simulink library "WECSim_Lib_Body_Elements"  (R2020b)
settings: Solver=VariableStepAuto  StartTime=0.0  StopTime=10.0  RelTol=1e-3
undefined symbols (not defined in the file or in its folder): body, simu, waves, X, Y, Z
libraries: nesl_utility x22, sm_lib x16, $bdroot x9, vrlib x3
(part 3 of 5)

== system WECSim_Lib_Body_Elements/Rigid Body/Hydrodynamic Body/B2B Subsystem/B2B ==
  CrossCoupling : Subsystem  mask{body=body}
      mask prompts: body "Body Number"
      mask help: This is used to
      mask init:
      | %In the initialization tab we place the code modifying the block
      | 
      | cb = gcb;
      | % position of initial blocks
      | set_param([cb '/vel1'],'Position',[200 1*50 240 (1*50+30)])
      | set_param([cb '/Mux1'], 'Position',[375 40 380 90])
      | set_param([cb '/vel'], 'Position',[410 59 440 71])
      | set_param([cb '/acc1'],'Position',[600 1*50 640 (1*50+30)])
      | set_param([cb '/Mux2'], 'Position',[775 40 780 90])
      | set_param([cb '/acc'], 'Position',[810 59 840 71])
      | set_param([cb '/Transport Delay1'], 'Position', [650 1*50 690 (1*50+30)])
      | 
      | % add/delete lines & blocks
      | newInputs = 0;
      | numbodies = body.total;
      | iBod = 2;
      | while iBod < 100
      |     try 
      |         find_system([cb,'/vel',num2str(iBod)],'Type','Block');
      |         if iBod > numbodies
      |             %delete 'From' blocks and lines if bodynumber > total bodies
      |             delete_line(cb,['vel',num2str(iBod),'/1'],['Mux',num2str(1),'/',num2str(iBod)])
      |             delete_line(cb,['acc',num2str(iBod),'/1'],['Transport Delay',num2str(iBod),'/1'])
      |             delete_line(cb,['Transport Delay',num2str(iBod),'/1'],['Mux',num2str(2),'/',num2str(iBod)])
      |             delete_block([cb '/vel',num2str(iBod)])
      |             delete_block([cb '/acc',num2str(iBod)])
      |             delete_block([cb '/Transport Delay',num2str(iBod)])
      |         end
      |     catch
      |         %set number of outputs for 'Mux Creator' blocks 
      |         if newInputs==0
      |             set_param([cb,'/Mux1'],'Inputs',num2str(numbodies))
      |             set_param([cb,'/Mux2'],'Inputs',num2str(numbodies))
      |         end
      |         if iBod <= numbodies
      |             newInputs = newInputs + 1;
      |             %add velocity 'From' block
      |             add_block('simulink/Signal Routing/From', [cb,'/vel',num2str(iBod)],'MakeNameUnique', 'on',...
      |             'Position',[200 iBod*50 240 (iBod*50+30)], 'BackgroundColor','green')
      |             h=[cb,'/vel',num2str(iBod)];
      |             responseName=['vel' num2str(iBod)];
      |             set_param(h,'GotoTag',responseName);
      |             %add acceleration 'From' block
      |             add_block('simulink/Signal Routing/From', [cb,'/acc',num2str(iBod)],'MakeNameUnique', 'on',...
      |             'Position',[600 iBod*50 640 (iBod*50+30)], 'BackgroundColor','green')
      |             h=[cb,'/acc',num2str(iBod)];
      |             responseName=['acc' num2str(iBod)];
      |             set_param(h,'GotoTag',responseName);
      |             % add transport delay block 
      |             add_block('simulink/Continuous/Transport Delay', [cb,'/Transport Delay',num2str(iBod)],'MakeNameUnique', 'on',...
      |             'Position',[650 iBod*50 690 (iBod*50+30)])
      |             h=[cb,'/Transport Delay',num2str(iBod)];
      |             set_param(h,'DelayTime',num2str(10e-8));
      |             %add lines
      |             add_line(cb,['vel',num2str(iBod),'/1'],['Mux',num2str(1),'/',num2str(iBod)])
      |             add_line(cb,['acc',num2str(iBod),'/1'],['Transport Delay',num2str(iBod),'/1'])
      |             add_line(cb,['Transport Delay',num2str(iBod),'/1'],['Mux',num2str(2),'/',num2str(iBod)])
      |             
      |         else
      |             break
      |         end
      |     end
      |     iBod = iBod + 1;
      | end
      mask Callback body: %customsat_callback('input',gcb)
      mask DialogControl DescGroupVar Prompt: Coupling Block
      mask DialogControl DescTextVar Prompt: This block transfers the velocity and acceleration vectors between bodies allowing for the coupled hydrodynamic forces to be calculated.  This block should not be included if there is only one body or if the hydrodynamic coupling parameter is set to 'No' in the rigid body block.
  vel : Outport
  acc : Outport  Port=2
  wires:
  CrossCoupling/1(vel) -> vel/1
  CrossCoupling/2(acc) -> acc/1

== system WECSim_Lib_Body_Elements/Rigid Body/Hydrodynamic Body/B2B Subsystem/noB2B ==
  vel_in : Inport
  acc_in : Inport  Port=2
  vel : Outport
  acc : Outport  Port=2
  wires:
  vel_in/1 -> vel/1  "x"
  acc_in/1 -> acc/1

== system WECSim_Lib_Body_Elements/Rigid Body/Hydrodynamic Body/Hydrostatic Restoring Force Calculation/Linear and Nonlinear Restoring Force Variant Subsystem ==
  note: If simu.nlHydro == 0, use the linear force option.
      | If simu.nlHydro > 0, use the nonlinear force option.
  note: 1) Add Subsystem or Model blocks as valid variant choices.
      | 2) You cannot connect blocks at this level. At simulation, connectivity is automatically
      | determined, based on the active variant and port name matching.
  In1 : Inport
  In2 : Inport  Port=2
  Linear Hydrostatic Restoring Force : Subsystem  VariantControl=sv_b1_linearHydro
  Nonlinear Hydrostatic Restoring Force : Subsystem  VariantControl=sv_b1_nonlinearHydro
  Out1 : Outport

== system WECSim_Lib_Body_Elements/Rigid Body/Hydrodynamic Body/Morison Element and Viscous Damping Force Calculation/Morison Element Variant Subsystem ==
  note: If body.morisonElement.option == 0, Morison element is off and the Morison force is 0
      | If body.morisonElement.option == 1 | 2, Morison element is on
  note: 1) Add Subsystem or Model blocks as valid variant choices.
      | 2) You cannot connect blocks at this level. At simulation, connectivity is automatically
      | determined, based on the active variant and port name matching.
  displacement : Inport
  velocity : Inport  Port=2
  acceleration : Inport  Port=3
  time : Inport  Port=4
  Morison Element Off : Subsystem  VariantControl=sv_b1_MEOff
  Morison Element On : Subsystem  Variant=on  VariantControl=sv_b1_MEOn
  morison_force : Outport

== system WECSim_Lib_Body_Elements/Rigid Body/Hydrodynamic Body/Nonlinear Wave Elevation/Linear or Instantaneous Free Surface ==
  note: If simu.nlHydro < 2, use the mean water free surface.
      | If simu.nlHydro == 2, use the instantaneous water free surface
  note: 1) Add Subsystem or Model blocks as valid variant choices.
      | 2) You cannot connect blocks at this level. At simulation, connectivity is automatically
      | determined, based on the active variant and port name matching.
  In1 : Inport
  In2 : Inport  Port=2
  Instantaneous Water Free Surface : Subsystem  VariantControl=sv_b1_instFS
  Mean Water Free Surface : Subsystem  VariantControl=sv_b1_meanFS
  Out1 : Outport

== system WECSim_Lib_Body_Elements/Rigid Body/Hydrodynamic Body/Structure/Motion Sensor ==
  note: Measures the position, velocity, and acceleration of the follower (F) frame relative to the base (B) frame.
      | Ouputs a bus of 3 signals, each signal is a vector length 6.
  Bus Creator : BusCreator  Inputs=3
  Mux : Mux
  Mux1 : Mux  Inputs=6
  Mux2 : Mux  Inputs=6
  PS-Simulink Converter{,1..15} (16 alike) : nesl_utility/PS-Simulink Converter  PhysicalDomain=network_engine_domain  SubClassName=ps_output  LeftPortType=input  RightPortType=output  PseudoPeriodic=off  Frequencies=[]  VectorFormat=1-D array  Unit=1  AffineConversion=off
  Transform Sensor : sm_lib/Frames and Transforms/Transform Sensor  MeasurementFrame=World  RotationSequence=XYX  SenseAngle=off  SenseAxis=off  SenseQ=on  SenseR=off  SenseRotationSequence=off  SenseOmegaX=on  SenseOmegaY=on  SenseOmegaZ=on  SenseOmega=off  SenseQDot=off  SenseRDot=off  SenseRotationSequenceDot=off  SenseAlphaX=on  SenseAlphaY=on  SenseAlphaZ=on  SenseAlpha=off  SenseQDDot=off  SenseRDDot=off  SenseX=on  SenseY=on  SenseZ=on  SenseXYZ=off  SenseRad=off  SenseAzim=off  SenseDist=off  SenseInc=off  SenseXDot=on  SenseYDot=on  SenseZDot=on  SenseXYZDot=off  SenseRadDot=off  SenseAzimDot=off  SenseDistDot=off  SenseIncDot=off  SenseXDDot=on  SenseYDDot=on  SenseZDDot=on  SenseXYZDDot=off  SenseRadDDot=off  SenseAzimDDot=off  SenseDistDDot=off  SenseIncDDot=off
  quaternion2EulXYZ : MATLAB Function  TreatAsAtomicUnit=on
  F : PMIOPort  Side=Right
  B : PMIOPort  Port=2  Side=Left
  Response : Outport
  wires:
  Bus Creator/1 -> Response/1
  PS-Simulink Converter15/1 -> Mux2/3  "az"
  PS-Simulink Converter3/1 -> Mux1/6  "omegaz"
  PS-Simulink Converter11/1 -> Mux1/2  "vy"
  PS-Simulink Converter2/1 -> Mux1/5  "omegay"
  PS-Simulink Converter1/1 -> Mux1/4  "omegax"
  PS-Simulink Converter6/1 -> Mux2/6  "alphaz"
  PS-Simulink Converter5/1 -> Mux2/5  "alphay"
  PS-Simulink Converter9/1 -> Mux/3  "z"
  PS-Simulink Converter8/1 -> Mux/2  "y"
  PS-Simulink Converter7/1 -> Mux/1  "x"
  Mux2/1 -> Bus Creator/3  "acc"
  Mux1/1 -> Bus Creator/2  "vel"
  Mux/1 -> Bus Creator/1  "disp"
  PS-Simulink Converter14/1 -> Mux2/2  "ay"
  PS-Simulink Converter13/1 -> Mux2/1  "ax"
  PS-Simulink Converter12/1 -> Mux1/3  "vz"
  PS-Simulink Converter10/1 -> Mux1/1  "vx"
  PS-Simulink Converter4/1 -> Mux2/4  "alphax"
  quaternion2EulXYZ/1(E) -> Mux/4
  PS-Simulink Converter/1 -> quaternion2EulXYZ/1(Q)
  connections:
  B/RConn1 -- Transform Sensor/LConn1
  Transform Sensor/RConn1 -- F/RConn1
  PS-Simulink Converter15/LConn1 -- Transform Sensor/RConn17
  Transform Sensor/RConn2 -- PS-Simulink Converter/LConn1
  PS-Simulink Converter1/LConn1 -- Transform Sensor/RConn3
  Transform Sensor/RConn4 -- PS-Simulink Converter2/LConn1
  PS-Simulink Converter3/LConn1 -- Transform Sensor/RConn5
  Transform Sensor/RConn6 -- PS-Simulink Converter4/LConn1
  PS-Simulink Converter5/LConn1 -- Transform Sensor/RConn7
  Transform Sensor/RConn8 -- PS-Simulink Converter6/LConn1
  PS-Simulink Converter7/LConn1 -- Transform Sensor/RConn9
  Transform Sensor/RConn10 -- PS-Simulink Converter8/LConn1
  PS-Simulink Converter9/LConn1 -- Transform Sensor/RConn11
  PS-Simulink Converter10/LConn1 -- Transform Sensor/RConn12
  Transform Sensor/RConn13 -- PS-Simulink Converter11/LConn1
  PS-Simulink Converter12/LConn1 -- Transform Sensor/RConn14
  PS-Simulink Converter13/LConn1 -- Transform Sensor/RConn15
  Transform Sensor/RConn16 -- PS-Simulink Converter14/LConn1

== system WECSim_Lib_Body_Elements/Rigid Body/Hydrodynamic Body/Variable Hydrodynamics Control/Variable Hydrodynamics Subsystem ==
  note: 1) Add Subsystem or Model blocks as valid variant choices.
      | 2) You cannot connect blocks at this level. At simulation, connectivity is automatically
      | determined, based on the active variant and port name matching.
  all_hydroForce : Inport
  noVariableHydro : Subsystem  VariantControl=sv_b1_noVariableHydro
  variableHydro : Subsystem  VariantControl=sv_b1_variableHydro  mask{body=body}
      mask prompts: body "Body Number:"
      mask init: same as WECSim_Lib_Body_Elements/Flex Body/Variable Hydrodynamics Control/Variable Hydrodynamics Subsystem/variableHydro
  selected_hydroForce : Outport

== system WECSim_Lib_Body_Elements/Rigid Body/Hydrodynamic Body/Wave Diffraction and Excitation Force Calculation/FexcInputs ==
  Time : Inport
  Displacement : Inport  Port=2
  WaveElv : Inport  Port=3
  body_hydroForce : Inport  Port=4
  Out1 : Outport
  Out2 : Outport  Port=2
  Out3 : Outport  Port=3
  Out4 : Outport  Port=4
  wires:
  WaveElv/1 -> Out3/1
  Time/1 -> Out1/1
  Displacement/1 -> Out2/1
  body_hydroForce/1 -> Out4/1

== system WECSim_Lib_Body_Elements/Rigid Body/Hydrodynamic Body/Wave Diffraction and Excitation Force Calculation/Linear Wave Excitation Force Variant Subsystem ==
  note: No wave includes wave.type == 'noWave' or 'noWaveCIC'
      | Regular wave includes wave.type == 'regular' or 'regularCIC'
      | Irregular wave includes wave.type == 'irregular' or 'spectrumImport'
  note: 1) Add Subsystem or Model blocks as valid variant choices.
      | 2) You cannot connect blocks at this level. At simulation, connectivity is automatically
      | determined, based on the active variant and port name matching.
  Time : Inport
  Displacement : Inport  Port=2
  body_hydroForce : Inport  Port=3
  Irregular Wave Excitation Force : Subsystem  VariantControl=sv_irregularWaves_b1
  Irregular Wave NonLinearYaw : Subsystem  VariantControl=sv_irregularWavesYaw_b1
  Irregular Wave Full Direction : Subsystem  VariantControl=sv_fullDirIrregularWaves_b1
  No Wave Excitation Force : Subsystem  VariantControl=sv_noWave
  Regular Wave Excitation Force : Subsystem  VariantControl=sv_regularWaves_b1
  Regular Wave NonLinear Yaw : Subsystem  VariantControl=sv_regularWavesYaw_b1
  User Defined Wave Excitation Force : Subsystem  VariantControl=sv_udfWaves
  Linear Excitation : Outport

== system WECSim_Lib_Body_Elements/Rigid Body/Hydrodynamic Body/Wave Diffraction and Excitation Force Calculation/Nonlinear FK Force Variant Subsystem ==
  note: If simu.nlHydro == 0, use No Nonlinear FroudeKrylov force option (nonlinear force is zero),
      | If simu.nlHydro > 0, use the Nonlinear FroudeKrylov force option,
  note: 1) Add Subsystem or Model blocks as valid variant choices.
      | 2) You cannot connect blocks at this level. At simulation, connectivity is automatically
      | determined, based on the active variant and port name matching.
  Time : Inport
  Displacement : Inport  Port=2
  WaveElv : Inport  Port=3
  No Nonlinear FroudeKrylov Force : Subsystem  VariantControl=sv_b1_linearHydro
  With Nonlinear FroudeKrylov Force : Subsystem  TreatAsAtomicUnit=on  SystemSampleTime=simu.nonlinearDt  VariantControl=sv_b1_nonlinearHydro
  Nonlinear Excitation : Outport

== system WECSim_Lib_Body_Elements/Rigid Body/Hydrodynamic Body/Wave Diffraction and Excitation Force Calculation/Ramp function ==
  note: The ramp function R, is a smooth function:
      | R = (sin(3*pi/2 + pi * t/Tr) + 1)/2 from t=0 to t=Tr
  Time : Inport
  Add1 : Sum
  Add2 : Sum
  Constant1 : Constant  Value=1/2
  Constant2 : Constant
  Constant3 : Constant  Value=3*pi/2
  Constant4 : Constant  Value=pi
  Divide : Product  Inputs=*/
  Product1 : Product
  Product2 : Product
  Ramp Time : Constant  Value=simu.rampTime
  Sine Wave Function : Sin  TimeSource=Use external signal  SampleTime=0
  R : Outport
  wires:
  Constant1/1 -> Product1/2
  Sine Wave Function/1 -> Add1/2
  Time/1 -> Product2/1
  Product2/1 -> Add2/1
  Add2/1 -> Sine Wave Function/1
  Constant4/1 -> Divide/1
  Add1/1 -> Product1/1
  Divide/1 -> Product2/2  "frequency"
  Ramp Time/1 -> Divide/2  "t_ramp"
  Constant3/1 -> Add2/2  "phase"
  Constant2/1 -> Add1/1
  Product1/1 -> R/1

== system WECSim_Lib_Body_Elements/Rigid Body/Hydrodynamic Body/Wave Diffraction and Excitation Force Calculation/Second Order Excitation Force Variant Subsystem ==
  note: 1) Add Subsystem or Model blocks as valid variant choices.
      | 2) You cannot connect blocks at this level. At simulation, connectivity is automatically
      | determined, based on the active variant and port name matching.
  Time : Inport
  body_hydroForce : Inport  Port=2
  displacement : Inport  Port=3
  No Second Order Excitation Force : Subsystem  VariantControl=sv_b1_noSecondOrderExt
  With Second Order Excitation Force : Subsystem  VariantControl=sv_b1_secondOrderExt
  Second Order Excitation : Outport

== system WECSim_Lib_Body_Elements/Rigid Body/Hydrodynamic Body/Wave Radiation Forces Calculation/SS CI and Constant-Damping-CoeVariant Subsystem ==
  note: If the wave type is 'noWave' or 'regular' use constant coefficients.
      | If another wave type and simu.Calc ~= 1, use convolution integral calculation
      | If another wave type and simu.Calc == 1, use the state space calculation
      | If another wave type and simu.FIR == 1, use the FIR filter calculation
  note: 1) Add Subsystem or Model blocks as valid variant choices.
      | 2) You cannot connect blocks at this level. At simulation, connectivity is automatically
      | determined, based on the active variant and port name matching.
  velocity : Inport
  Constant Coefficients : Subsystem  VariantControl=sv_constantCoeff
  Convolution Integral Calculation : Subsystem  VariantControl=sv_convolution
  FIR Filter Calculation : Subsystem  VariantControl=sv_FIR
  "State-Space Calculation " : Subsystem  VariantControl=sv_stateSpace
  Out1 : Outport

== system WECSim_Lib_Body_Elements/Rigid Body/Hydrodynamic Body/Yaw Kinematic Transforms/No B2B ==
  note: If body.yaw.option == 1, interpolate the BEM coefficients to account for the effective change in the incoming wave direction.
  dispGlobal : Inport
  velGlobal : Inport  Port=2
  accGlobal : Inport  Port=3
  Constant : Constant  Value=body.yaw.option
  Yaw Kinematic Transforms : MATLAB Function  TreatAsAtomicUnit=on
  dispLoc : Outport
  velLoc : Outport  Port=2
  accLoc : Outport  Port=3
  wires:
  dispGlobal/1 -> Yaw Kinematic Transforms/2(dispGlobal)
  velGlobal/1 -> Yaw Kinematic Transforms/3(velGlobal)
  accGlobal/1 -> Yaw Kinematic Transforms/4(accGlobal)
  Constant/1 -> Yaw Kinematic Transforms/1(yaw)
  Yaw Kinematic Transforms/2(velLoc) -> velLoc/1
  Yaw Kinematic Transforms/1(dispLoc) -> dispLoc/1
  Yaw Kinematic Transforms/3(accLoc) -> accLoc/1

== system WECSim_Lib_Body_Elements/Rigid Body/Hydrodynamic Body/Yaw Kinematic Transforms/With B2B ==
  note: If body.yaw.option == 1, interpolate the BEM coefficients to account for the effective change in the incoming wave direction.
  dispGlobal : Inport
  velGlobal : Inport  Port=2
  accGlobal : Inport  Port=3
  Constant : Constant  Value=body.yaw.option
  Yaw Kinematic Transforms : MATLAB Function  TreatAsAtomicUnit=on
  dispLoc : Outport
  velLoc : Outport  Port=2
  accLoc : Outport  Port=3
  wires:
  Constant/1 -> Yaw Kinematic Transforms/1(yaw)
  Yaw Kinematic Transforms/1(dispLoc) -> dispLoc/1
  Yaw Kinematic Transforms/2(velLoc) -> velLoc/1
  Yaw Kinematic Transforms/3(accLoc) -> accLoc/1
  dispGlobal/1 -> Yaw Kinematic Transforms/2(dispGlobal)
  velGlobal/1 -> Yaw Kinematic Transforms/3(velGlobal)
  accGlobal/1 -> Yaw Kinematic Transforms/4(accGlobal)

== system WECSim_Lib_Body_Elements/Flex Body/Hydrostatic Restoring Force Calculation/Hydrostatic Restoring Force Calculation/Linear and Nonlinear Restoring Force Variant Subsystem/Linear Hydrostatic Restoring Force ==
  note: The total hydrostatic restoring force is due to a linear stiffness, the vertical buoyancy force (gravity - buoyancy) and a rotational buoyancy force if the center of gravity is not aligned with the center of buoyancy.
      |
      | F_restoring = F_linearRestoringStiffness + F_NetBuoyancy
      |
      | F_linear restoring = hydrostatic restoring coefficient * displacement
      | F_NetBuoyancy = F_gravity - F_buoyancy + F_rotational_buoyancy
      |
      | F_rotational_buoyancy = (cb-cg) x F_buoyancy
      | F_buoyancy = rho*g*V_0
      | F_gravity = m*g
  In1 : Inport
  Add : Sum
  Bus Selector1 : BusSelector  OutputSignals=mass,volume,centerBuoyancy,linearHydroRestCoef
  Net Buoyancy Force : Subsystem
  Product2 : Product  Multiplication=Matrix(*)
  Out1 : Outport
  wires:
  Net Buoyancy Force/1(F_NetBuoyancy) -> Add/1  "Net buoyancy force"
  Bus Selector1/1 -> Net Buoyancy Force/1(Body Mass)  "<mass>"
  Bus Selector1/4 -> Product2/1  "<linearHydroRestCoef>"
  Bus Selector1/2 -> Net Buoyancy Force/2(Volume)  "<volume>"
  [body1_hydroForce] -> Bus Selector1/1
  Bus Selector1/3 -> Net Buoyancy Force/3(Center of Buoyancy)  "<centerBuoyancy>"
  Product2/1 -> Add/2  "Linear Restoring Force"
  In1/1 -> Product2/2  "x"
  Add/1 -> Out1/1  "F_Restoring"

== system WECSim_Lib_Body_Elements/Flex Body/Hydrostatic Restoring Force Calculation/Hydrostatic Restoring Force Calculation/Linear and Nonlinear Restoring Force Variant Subsystem/Nonlinear Hydrostatic Restoring Force ==
  In1 : Inport
  In2 : Inport  Port=2
  Add : Sum
  Bus Selector1 : BusSelector  OutputSignals=storage.mass,volume,centerBuoyancy,linearHydroRestCoef
  Center of Gravity : Constant  Value=body.centerGravity
  Gravity : Constant  Value=simu.gravity
  Mux1 : Mux  Inputs=2
  Net Buoyancy Force : Subsystem
  Product2 : Product  Multiplication=Matrix(*)
  Rate Transition : RateTransition
  Rate Transition1 : RateTransition
  Restoring Forces : MATLAB Function  TreatAsAtomicUnit=on  SystemSampleTime=simu.nonlinearDt
  STL areas : Constant  Value=body.geometry.area
  STL centers : Constant  Value=body.geometry.center
  STL normal vectors : Constant  Value=body.geometry.norm
  Selector : Selector  InputPortWidth=body.dof  IndexOptions=Index vector (dialog)  Indices=[7:body.dofEnd]  OutputSizes=1
  To Workspace1 : ToWorkspace  VariableName=body1_hspressure_out  SaveFormat=Structure With Time  SampleTime=-1
      settings: Decimation=round(simu.dtOut/simu.dt,0)
  Water Density : Constant  Value=simu.rho
  Out1 : Outport
  wires:
  [body1_hydroForce] -> Bus Selector1/1
  Center of Gravity/1 -> Restoring Forces/8(cg)
  Gravity/1 -> Restoring Forces/7(g)  "g"
  Water Density/1 -> Restoring Forces/6(rho)
  STL normal vectors/1 -> Restoring Forces/4(tnorm)
  STL centers/1 -> Restoring Forces/3(center)
  In2/1 -> Restoring Forces/2(elv)
  STL areas/1 -> Restoring Forces/5(area)
  Restoring Forces/2(p) -> Rate Transition1/1
  Rate Transition1/1 -> To Workspace1/1
  Restoring Forces/1(f) -> Rate Transition/1
  Rate Transition/1 -> Mux1/1
  Mux1/1 -> Out1/1
  Add/1 -> Selector/1  "F_Restoring"
  Bus Selector1/4 -> Product2/1  "<linearHydroRestCoef>"
  Bus Selector1/1 -> Restoring Forces/9(mass), Net Buoyancy Force/1(Body Mass)  "<mass>"
  Net Buoyancy Force/1(F_NetBuoyancy) -> Add/1  "Net buoyancy force"
  Bus Selector1/3 -> Net Buoyancy Force/3(Center of Buoyancy)  "<centerBuoyancy>"
  In1/1 -> Product2/2, Restoring Forces/1(x)  "x"
  Bus Selector1/2 -> Net Buoyancy Force/2(Volume)  "<volume>"
  Product2/1 -> Add/2  "Linear Restoring Force"
  Selector/1 -> Mux1/2

== system WECSim_Lib_Body_Elements/Flex Body/Wave Diffraction and Excitation Force Calculation/Wave Diffraction and Excitation Force Calculation/Linear Wave Excitation Force Variant Subsystem/Irregular Wave Excitation Force ==
  note: Calculates the wave force, F_wave, for the case of Irregular Waves.
      |
      | The total force is the combination of the real excitation force, imaginary excitation force, and real part of the mean drift force (fExt.md)
      |
      | F_wave =   sum(A * cos(w * t) * Re{Fext(i)}
      |                            -  A * sin(w * t) * Im{Fext(i)}
      |                            + A * Re(Fext.md(i))
      |                            )
      |
      | where i = each frequency bin
  Time : Inport
  Displacement : Inport  Port=2
  body_hydroForce : Inport  Port=3
  Add : Sum  Inputs=+-
  Bus Selector : BusSelector  OutputSignals=fExt.re,fExt.im,fExt.md
  Center of Gravity : Constant  Value=body.centerGravity
  Constant : Constant  Value=zeros(1,body.dof-3)
  Displacement Phase Enable1 : Constant  Value=body.largeXYDisplacement.option
  Frequency Spacing Delta Omega : Constant  Value=Nwave.dOmega  VectorParams1D=off
  MATLAB Function : MATLAB Function  TreatAsAtomicUnit=on
  MATLAB Function2 : MATLAB Function  TreatAsAtomicUnit=on
  Mux : Mux  Inputs=2
  Random Phase : Constant  Value=Nwave.phase  VectorParams1D=off
  Selector : Selector  IndexOptions=Index vector (dialog)  Indices=[1 2]  OutputSizes=1
  Sum : Sum  Inputs=|++
  Wave Frequency : Constant  Value=Nwave.omega  VectorParams1D=off
  Wave Frequency1 : Constant  Value=Nwave.omega  VectorParams1D=off
  Wave Number1 : Constant  Value=Nwave.wavenumber
  Wave Spectrum : Constant  Value=Nwave.amplitude  VectorParams1D=off
  Wave direction spread : Constant  Value=Nwave.spread  VectorParams1D=off
  Wave direction1 : Constant  Value=Nwave.direction  VectorParams1D=off
  Linear Excitation : Outport
  wires:
  Bus Selector/1 -> MATLAB Function/3(fExtRE)  "<re>"
  body_hydroForce/1 -> Bus Selector/1
  Wave direction1/1 -> MATLAB Function2/5(direction), MATLAB Function/8(WaveDir)
  Wave Number1/1 -> MATLAB Function2/4(wavenumber)
  Selector/1 -> MATLAB Function2/1(disp)
  Displacement Phase Enable1/1 -> MATLAB Function2/2(enable)
  Wave Frequency1/1 -> MATLAB Function2/3(frequency)
  Random Phase/1 -> Sum/1
  Sum/1 -> MATLAB Function/5(phaseRand)
  MATLAB Function2/1(dispPhase) -> Sum/2
  Bus Selector/3 -> MATLAB Function/10(fExtMD)  "<md>"
  Wave direction spread/1 -> MATLAB Function/9(spread)
  Frequency Spacing Delta Omega/1 -> MATLAB Function/6(dw)
  Time/1 -> MATLAB Function/7(time)
  Wave Spectrum/1 -> MATLAB Function/1(A)
  Bus Selector/2 -> MATLAB Function/4(fExtIM)  "<im>"
  Wave Frequency/1 -> MATLAB Function/2(w)
  MATLAB Function/1(Fext) -> Linear Excitation/1
  Displacement/1 -> Add/1  "t"
  Mux/1 -> Add/2
  Constant/1 -> Mux/2
  Center of Gravity/1 -> Mux/1  "cg"
  Add/1 -> Selector/1  "x_cg"

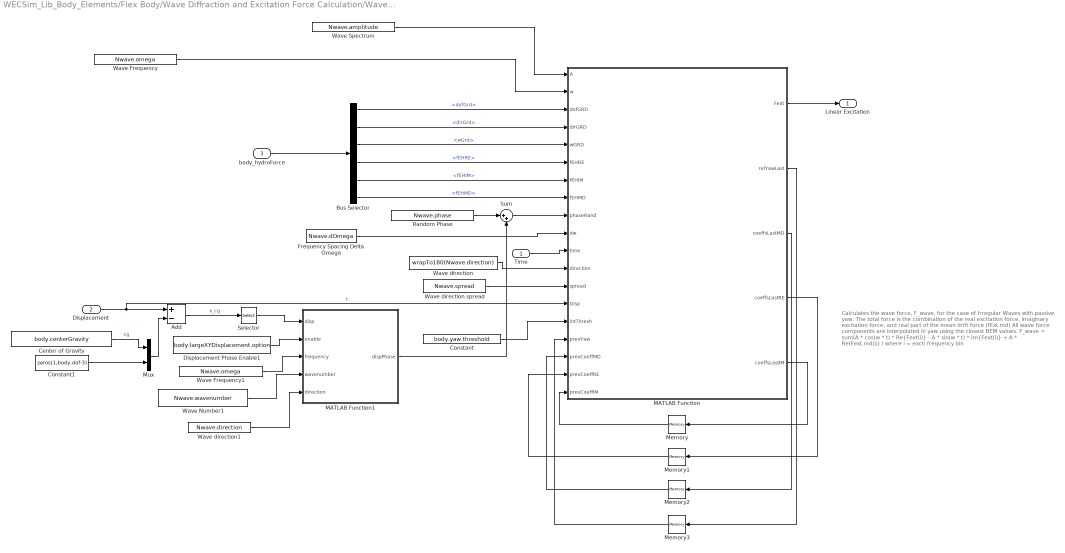
== system WECSim_Lib_Body_Elements/Flex Body/Wave Diffraction and Excitation Force Calculation/Wave Diffraction and Excitation Force Calculation/Linear Wave Excitation Force Variant Subsystem/Irregular Wave NonLinearYaw ==
  note: Calculates the wave force, F_wave, for the case of Irregular Waves with passive yaw.
      |
      | The total force is the combination of the real excitation force, imaginary excitation force, and real part of the mean drift force (fExt.md)
      |
      | All wave force components are interpolated in yaw using the closest BEM values.
      |
      | F_wave =   sum(A * cos(w * t) * Re{Fext(i)}
      |                            -  A * sin(w * t) * Im{Fext(i)}
      |                            + A * Re(Fext.md(i))
      |                            )
      |
      | where i = each frequency bin
  Time : Inport
  Displacement : Inport  Port=2
  body_hydroForce : Inport  Port=3
  Add : Sum  Inputs=+-
  Bus Selector : BusSelector  OutputSignals=fExt.dofGrd,fExt.dirGrd,fExt.wGrd,fExt.fEHRE,fExt.fEHIM,fExt.fEHMD
  Center of Gravity : Constant  Value=body.centerGravity
  Constant : Constant  Value=body.yaw.threshold
  Constant1 : Constant  Value=zeros(1,body.dof-3)
  Displacement Phase Enable1 : Constant  Value=body.largeXYDisplacement.option
  Frequency Spacing Delta Omega : Constant  Value=Nwave.dOmega  VectorParams1D=off
  MATLAB Function : MATLAB Function  TreatAsAtomicUnit=on
  MATLAB Function1 : MATLAB Function  TreatAsAtomicUnit=on
  Memory{,1..3} (4 alike) : Memory  InheritSampleTime=on  LinearizeAsDelay=on
  Mux : Mux  Inputs=2
  Random Phase : Constant  Value=Nwave.phase  VectorParams1D=off
  Selector : Selector  IndexOptions=Index vector (dialog)  Indices=[1 2]  OutputSizes=1
  Sum : Sum  Inputs=|++
  Wave Frequency : Constant  Value=Nwave.omega  VectorParams1D=off
  Wave Frequency1 : Constant  Value=Nwave.omega  VectorParams1D=off
  Wave Number1 : Constant  Value=Nwave.wavenumber
  Wave Spectrum : Constant  Value=Nwave.amplitude  VectorParams1D=off
  Wave direction : Constant  Value=wrapTo180(Nwave.direction)  VectorParams1D=off
  Wave direction spread : Constant  Value=Nwave.spread  VectorParams1D=off
  Wave direction1 : Constant  Value=Nwave.direction  VectorParams1D=off
  Linear Excitation : Outport
  wires:
  Bus Selector/5 -> MATLAB Function/7(fEHIM)  "<fEHIM>"
  Bus Selector/1 -> MATLAB Function/3(dofGRD)  "<dofGrd>"
  body_hydroForce/1 -> Bus Selector/1
  MATLAB Function1/1(dispPhase) -> Sum/2
  Wave direction1/1 -> MATLAB Function1/5(direction)
  Wave Number1/1 -> MATLAB Function1/4(wavenumber)
  Selector/1 -> MATLAB Function1/1(disp)
  Displacement Phase Enable1/1 -> MATLAB Function1/2(enable)
  Wave Frequency1/1 -> MATLAB Function1/3(frequency)
  Sum/1 -> MATLAB Function/9(phaseRand)
  Random Phase/1 -> Sum/1
  Time/1 -> MATLAB Function/11(time)
  Wave direction spread/1 -> MATLAB Function/13(spread)
  Bus Selector/6 -> MATLAB Function/8(fEHMD)  "<fEHMD>"
  Wave Spectrum/1 -> MATLAB Function/1(A)
  Wave Frequency/1 -> MATLAB Function/2(w)
  Memory/1 -> MATLAB Function/19(prevCoeffIM)
  Bus Selector/4 -> MATLAB Function/6(fEHRE)  "<fEHRE>"
  MATLAB Function/3(coeffsLastMD) -> Memory2/1
  Constant/1 -> MATLAB Function/15(intThresh)
  Memory3/1 -> MATLAB Function/16(prevYaw)
  MATLAB Function/5(coeffsLastIM) -> Memory/1
  Wave direction/1 -> MATLAB Function/12(direction)
  Frequency Spacing Delta Omega/1 -> MATLAB Function/10(dw)
  Bus Selector/2 -> MATLAB Function/4(dirGRD)  "<dirGrd>"
  Bus Selector/3 -> MATLAB Function/5(wGRD)  "<wGrd>"
  Memory2/1 -> MATLAB Function/17(prevCoeffMD)
  MATLAB Function/2(relYawLast) -> Memory3/1
  MATLAB Function/4(coeffsLastRE) -> Memory1/1
  Memory1/1 -> MATLAB Function/18(prevCoeffRE)
  MATLAB Function/1(Fext) -> Linear Excitation/1
  Center of Gravity/1 -> Mux/1  "cg"
  Constant1/1 -> Mux/2
  Add/1 -> Selector/1  "x_cg"
  Displacement/1 -> MATLAB Function/14(Disp), Add/1  "t"
  Mux/1 -> Add/2

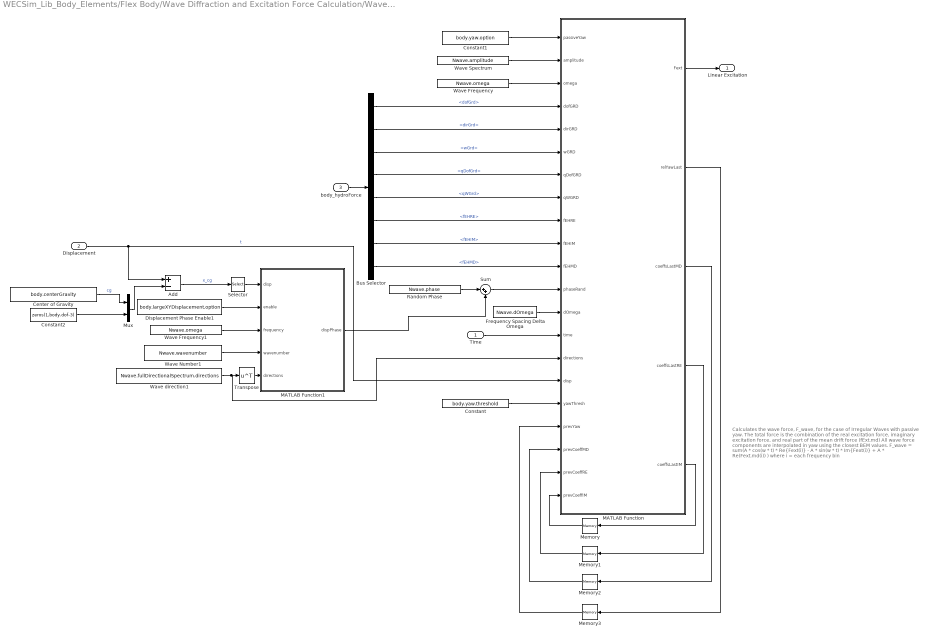
== system WECSim_Lib_Body_Elements/Flex Body/Wave Diffraction and Excitation Force Calculation/Wave Diffraction and Excitation Force Calculation/Linear Wave Excitation Force Variant Subsystem/Irregular Wave Full Direction ==
  note: Calculates the wave force, F_wave, for the case of Irregular Waves with passive yaw.
      |
      | The total force is the combination of the real excitation force, imaginary excitation force, and real part of the mean drift force (fExt.md)
      |
      | All wave force components are interpolated in yaw using the closest BEM values.
      |
      | F_wave =   sum(A * cos(w * t) * Re{Fext(i)}
      |                            -  A * sin(w * t) * Im{Fext(i)}
      |                            + A * Re(Fext.md(i))
      |                            )
      |
      | where i = each frequency bin
  Time : Inport
  Displacement : Inport  Port=2
  body_hydroForce : Inport  Port=3
  Add : Sum  Inputs=+-
  Bus Selector : BusSelector  OutputSignals=fExt.dofGrd,fExt.dirGrd,fExt.wGrd,fExt.qDofGrd,fExt.qWGrd,fExt.fEHRE,fExt.fEHIM,fExt.fEHMD
  Center of Gravity : Constant  Value=body.centerGravity
  Constant : Constant  Value=body.yaw.threshold
  Constant1 : Constant  Value=body.yaw.option
  Constant2 : Constant  Value=zeros(1,body.dof-3)
  Displacement Phase Enable1 : Constant  Value=body.largeXYDisplacement.option
  Frequency Spacing Delta Omega : Constant  Value=Nwave.dOmega  VectorParams1D=off
  MATLAB Function : MATLAB Function  TreatAsAtomicUnit=on
  MATLAB Function1 : MATLAB Function  TreatAsAtomicUnit=on
  Memory : Memory  InitialCondition=zeros(length(Nwave.fullDirectionalSpectrum.directions),length(Nwave.omega),6)  InheritSampleTime=on  LinearizeAsDelay=on
  Memory1 : Memory  InitialCondition=zeros(length(Nwave.fullDirectionalSpectrum.directions),length(Nwave.omega),6)  InheritSampleTime=on  LinearizeAsDelay=on
  Memory2 : Memory  InitialCondition=zeros(length(Nwave.fullDirectionalSpectrum.directions),length(Nwave.omega),6)  InheritSampleTime=on  LinearizeAsDelay=on
  Memory3 : Memory  InitialCondition=zeros(size(Nwave.fullDirectionalSpectrum.directions))  InheritSampleTime=on  LinearizeAsDelay=on
  Mux : Mux  Inputs=2
  Random Phase : Constant  Value=Nwave.phase  VectorParams1D=off
  Selector : Selector  IndexOptions=Index vector (dialog)  Indices=[1 2]  OutputSizes=1
  Sum : Sum  Inputs=|++
  Transpose : Math  Operator=transpose  SaturateOnIntegerOverflow=on
  Wave Frequency : Constant  Value=Nwave.omega  VectorParams1D=off
  Wave Frequency1 : Constant  Value=Nwave.omega  VectorParams1D=off
  Wave Number1 : Constant  Value=Nwave.wavenumber
  Wave Spectrum : Constant  Value=Nwave.amplitude  VectorParams1D=off
  Wave direction1 : Constant  Value=Nwave.fullDirectionalSpectrum.directions  VectorParams1D=off
  Linear Excitation : Outport
  wires:
  Wave Number1/1 -> MATLAB Function1/4(wavenumber)
  Bus Selector/5 -> MATLAB Function/8(qWGRD)  "<qWGrd>"
  MATLAB Function/3(coeffsLastMD) -> Memory2/1
  Memory2/1 -> MATLAB Function/19(prevCoeffMD)
  Wave Frequency/1 -> MATLAB Function/3(omega)
  MATLAB Function/4(coeffsLastRE) -> Memory1/1
  Bus Selector/4 -> MATLAB Function/7(qDofGRD)  "<qDofGrd>"
  Bus Selector/8 -> MATLAB Function/11(fEHMD)  "<fEHMD>"
  Constant/1 -> MATLAB Function/17(yawThresh)
  Time/1 -> MATLAB Function/14(time)
  Random Phase/1 -> Sum/1
  MATLAB Function/2(relYawLast) -> Memory3/1
  Bus Selector/2 -> MATLAB Function/5(dirGRD)  "<dirGrd>"
  Wave direction1/1 -> MATLAB Function/15(directions), Transpose/1
  Constant1/1 -> MATLAB Function/1(passiveYaw)
  Bus Selector/6 -> MATLAB Function/9(fEHRE)  "<fEHRE>"
  Wave Frequency1/1 -> MATLAB Function1/3(frequency)
  Selector/1 -> MATLAB Function1/1(disp)
  Memory1/1 -> MATLAB Function/20(prevCoeffRE)
  Displacement Phase Enable1/1 -> MATLAB Function1/2(enable)
  MATLAB Function/5(coeffsLastIM) -> Memory/1
  Memory3/1 -> MATLAB Function/18(prevYaw)
  Memory/1 -> MATLAB Function/21(prevCoeffIM)
  MATLAB Function/1(Fext) -> Linear Excitation/1
  Bus Selector/3 -> MATLAB Function/6(wGRD)  "<wGrd>"
  Bus Selector/1 -> MATLAB Function/4(dofGRD)  "<dofGrd>"
  Frequency Spacing Delta Omega/1 -> MATLAB Function/13(dOmega)
  body_hydroForce/1 -> Bus Selector/1
  Bus Selector/7 -> MATLAB Function/10(fEHIM)  "<fEHIM>"
  Sum/1 -> MATLAB Function/12(phaseRand)
  MATLAB Function1/1(dispPhase) -> Sum/2
  Wave Spectrum/1 -> MATLAB Function/2(amplitude)
  Transpose/1 -> MATLAB Function1/5(directions)
  Add/1 -> Selector/1  "x_cg"
  Center of Gravity/1 -> Mux/1  "cg"
  Mux/1 -> Add/2
  Constant2/1 -> Mux/2
  Displacement/1 -> Add/1, MATLAB Function/16(disp)  "t"

== system WECSim_Lib_Body_Elements/Flex Body/Wave Diffraction and Excitation Force Calculation/Wave Diffraction and Excitation Force Calculation/Linear Wave Excitation Force Variant Subsystem/No Wave Excitation Force ==
  Constant : Constant  Value=zeros(1,body.dof)
  Linear Excitation : Outport
  wires:
  Constant/1 -> Linear Excitation/1

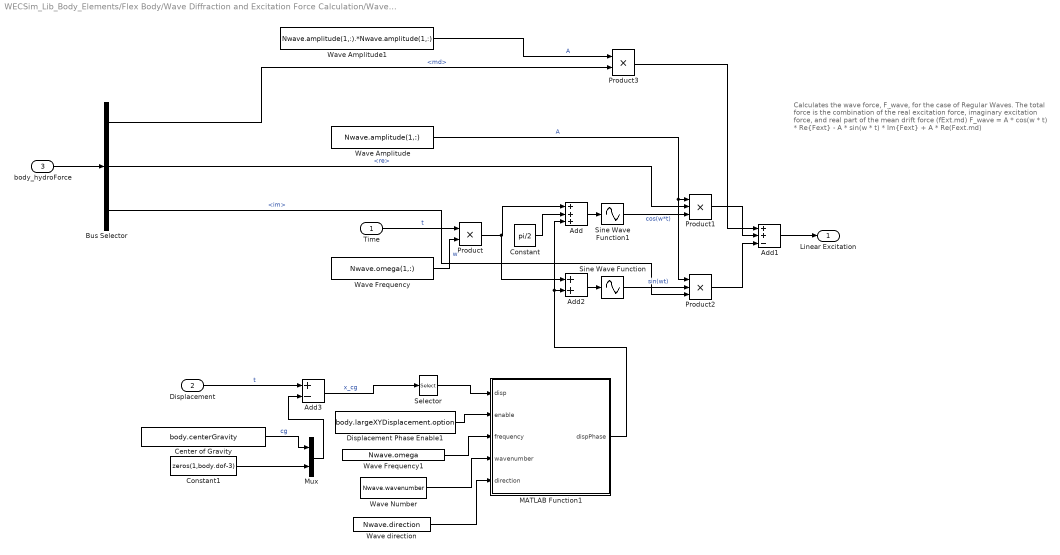
== system WECSim_Lib_Body_Elements/Flex Body/Wave Diffraction and Excitation Force Calculation/Wave Diffraction and Excitation Force Calculation/Linear Wave Excitation Force Variant Subsystem/Regular Wave Excitation Force ==
  note: Calculates the wave force, F_wave, for the case of Regular Waves.
      |
      | The total force is the combination of the real excitation force, imaginary excitation force, and real part of the mean drift force (fExt.md)
      |
      | F_wave =   A * cos(w * t) * Re{Fext}
      |                -  A * sin(w * t) * Im{Fext}
      |                + A * Re(Fext.md)
  Time : Inport
  Displacement : Inport  Port=2
  body_hydroForce : Inport  Port=3
  Add : Sum  Inputs=+++
  Add1 : Sum  Inputs=++-
  Add2 : Sum
  Add3 : Sum  Inputs=+-
  Bus Selector : BusSelector  OutputSignals=fExt.md,fExt.re,fExt.im
  Center of Gravity : Constant  Value=body.centerGravity
  Constant : Constant  Value=pi/2
  Constant1 : Constant  Value=zeros(1,body.dof-3)
  Displacement Phase Enable1 : Constant  Value=body.largeXYDisplacement.option
  MATLAB Function1 : MATLAB Function  TreatAsAtomicUnit=on
  Mux : Mux  Inputs=2
  Product : Product
  Product1 : Product  Inputs=3
  Product2 : Product  Inputs=3
  Product3 : Product
  Selector : Selector  IndexOptions=Index vector (dialog)  Indices=[1 2]  OutputSizes=1
  Sine Wave Function : Sin  TimeSource=Use external signal  SampleTime=0
  Sine Wave Function1 : Sin  TimeSource=Use external signal  SampleTime=0
  Wave Amplitude : Constant  Value=Nwave.amplitude(1,:)
  Wave Amplitude1 : Constant  Value=Nwave.amplitude(1,:).*Nwave.amplitude(1,:)
  Wave Frequency : Constant  Value=Nwave.omega(1,:)
  Wave Frequency1 : Constant  Value=Nwave.omega  VectorParams1D=off
  Wave Number : Constant  Value=Nwave.wavenumber
  Wave direction : Constant  Value=Nwave.direction  VectorParams1D=off
  Linear Excitation : Outport
  wires:
  Bus Selector/3 -> Product2/3  "<im>"
  Bus Selector/2 -> Product1/2  "<re>"
  Bus Selector/1 -> Product3/2  "<md>"
  body_hydroForce/1 -> Bus Selector/1
  Wave direction/1 -> MATLAB Function1/5(direction)
  Wave Number/1 -> MATLAB Function1/4(wavenumber)
  Wave Frequency1/1 -> MATLAB Function1/3(frequency)
  Selector/1 -> MATLAB Function1/1(disp)
  Add2/1 -> Sine Wave Function/1
  MATLAB Function1/1(dispPhase) -> Add2/2, Add/3
  Displacement Phase Enable1/1 -> MATLAB Function1/2(enable)
  Product3/1 -> Add1/1
  Wave Amplitude1/1 -> Product3/1  "A"
  Constant/1 -> Add/2
  Add/1 -> Sine Wave Function1/1
  Wave Amplitude/1 -> Product1/1, Product2/1  "A"
  Add1/1 -> Linear Excitation/1
  Product2/1 -> Add1/3
  Product1/1 -> Add1/2
  Sine Wave Function/1 -> Product2/2  "sin(wt)"
  Sine Wave Function1/1 -> Product1/3  "cos(w*t)"
  Product/1 -> Add/1, Add2/1
  Wave Frequency/1 -> Product/2  "w"
  Time/1 -> Product/1  "t"
  Displacement/1 -> Add3/1  "t"
  Constant1/1 -> Mux/2
  Center of Gravity/1 -> Mux/1  "cg"
  Add3/1 -> Selector/1  "x_cg"
  Mux/1 -> Add3/2

== system WECSim_Lib_Body_Elements/Flex Body/Wave Diffraction and Excitation Force Calculation/Wave Diffraction and Excitation Force Calculation/Linear Wave Excitation Force Variant Subsystem/Regular Wave NonLinear Yaw ==
  note: Calculates the wave force, F_wave, for the case of Regular Waves with passive yaw.
      |
      | The total force is the combination of the real excitation force, imaginary excitation force, and real part of the mean drift force (fExt.md)
      |
      | All wave force components are interpolated in yaw using the closest BEM values.
      |
      | F_wave =   A * cos(w * t) * Re{Fext}
      |                -  A * sin(w * t) * Im{Fext}
      |                + A * Re(Fext.md)
  Time : Inport
  Displacement : Inport  Port=2
  body_hydroForce : Inport  Port=3
  Add : Sum  Inputs=+-
  Bus Selector : BusSelector  OutputSignals=fExt.dofGrd,fExt.dirGrd,fExt.fEHRE,fExt.fEHIM,fExt.fEHMD
  Center of Gravity : Constant  Value=body.centerGravity
  Constant : Constant  Value=body.yaw.threshold
  Constant1 : Constant  Value=zeros(1,body.dof-3)
  Displacement Phase Enable1 : Constant  Value=body.largeXYDisplacement.option
  MATLAB Function1 : MATLAB Function  TreatAsAtomicUnit=on
  MATLAB Function3 : MATLAB Function  TreatAsAtomicUnit=on
  Memory{,1..3} (4 alike) : Memory  InheritSampleTime=on  LinearizeAsDelay=on
  Mux : Mux  Inputs=2
  Selector : Selector  IndexOptions=Index vector (dialog)  Indices=[1 2]  OutputSizes=1
  Wave Amplitude : Constant  Value=Nwave.amplitude(1,:)
  Wave Frequency : Constant  Value=Nwave.omega(1,:)
  Wave Frequency1 : Constant  Value=Nwave.omega  VectorParams1D=off
  Wave Number1 : Constant  Value=Nwave.wavenumber
  Wave direction : Constant  Value=wrapTo180(Nwave.direction)  VectorParams1D=off
  Wave direction1 : Constant  Value=Nwave.direction  VectorParams1D=off
  Linear Excitation : Outport
  wires:
  Bus Selector/3 -> MATLAB Function1/5(fEHRE)  "<fEHRE>"
  Bus Selector/4 -> MATLAB Function1/6(fEHIM)  "<fEHIM>"
  Bus Selector/1 -> MATLAB Function1/3(dofGRD)  "<dofGrd>"
  body_hydroForce/1 -> Bus Selector/1
  Wave Frequency1/1 -> MATLAB Function3/3(frequency)
  Selector/1 -> MATLAB Function3/1(disp)
  Displacement Phase Enable1/1 -> MATLAB Function3/2(enable)
  Wave Number1/1 -> MATLAB Function3/4(wavenumber)
  Wave direction1/1 -> MATLAB Function3/5(direction)
  MATLAB Function3/1(dispPhase) -> MATLAB Function1/12(phase)
  Time/1 -> MATLAB Function1/8(time)
  MATLAB Function1/1(Fext) -> Linear Excitation/1
  Wave Frequency/1 -> MATLAB Function1/2(w)  "w"
  MATLAB Function1/5(coeffsLastIM) -> Memory/1
  MATLAB Function1/2(relYawLast) -> Memory3/1
  MATLAB Function1/4(coeffsLastRE) -> Memory1/1
  Memory3/1 -> MATLAB Function1/13(prevYaw)
  Bus Selector/5 -> MATLAB Function1/7(fEHMD)  "<fEHMD>"
  Memory/1 -> MATLAB Function1/16(prevCoeffIM)
  Wave Amplitude/1 -> MATLAB Function1/1(A)  "A"
  MATLAB Function1/3(coeffsLastMD) -> Memory2/1
  Wave direction/1 -> MATLAB Function1/9(WaveDir)
  Memory1/1 -> MATLAB Function1/15(prevCoeffRE)
  Bus Selector/2 -> MATLAB Function1/4(dirGRD)  "<dirGrd>"
  Constant/1 -> MATLAB Function1/11(intThresh)
  Memory2/1 -> MATLAB Function1/14(prevCoeffMD)
  Mux/1 -> Add/2
  Add/1 -> Selector/1  "x_cg"
  Displacement/1 -> Add/1, MATLAB Function1/10(Disp)  "t"
  Constant1/1 -> Mux/2
  Center of Gravity/1 -> Mux/1  "cg"

== system WECSim_Lib_Body_Elements/Flex Body/Wave Diffraction and Excitation Force Calculation/Wave Diffraction and Excitation Force Calculation/Linear Wave Excitation Force Variant Subsystem/User Defined Wave Excitation Force ==
  note: Calculates the wave force, F_wave, for the case of User Defined Waves.
      |
      | F_wave = convolution calculation [1x6]
  InputWaveForceTimeHistory1 : FromWorkspace  VariableName=[Nwave.waveAmpTime(:,1),body.hydroForce.hf1.userDefinedFe]
  Linear Excitation : Outport
  wires:
  InputWaveForceTimeHistory1/1 -> Linear Excitation/1

== system WECSim_Lib_Body_Elements/Flex Body/Wave Diffraction and Excitation Force Calculation/Wave Diffraction and Excitation Force Calculation/Nonlinear FK Force Variant Subsystem/No Nonlinear FroudeKrylov Force ==
  Constant : Constant  Value=zeros(1,body.dof)
  Nonlinear Excitation : Outport
  wires:
  Constant/1 -> Nonlinear Excitation/1

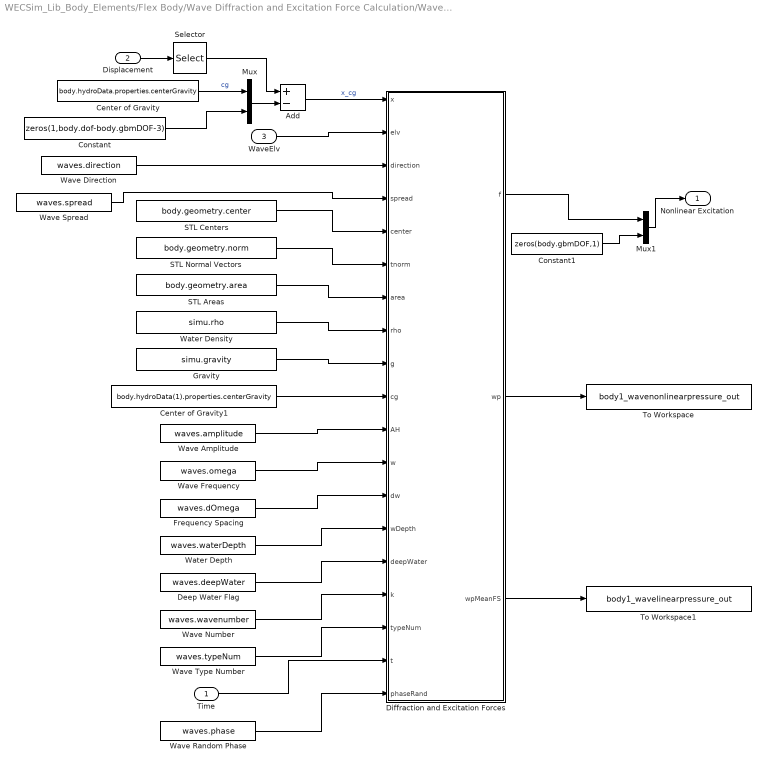
== system WECSim_Lib_Body_Elements/Flex Body/Wave Diffraction and Excitation Force Calculation/Wave Diffraction and Excitation Force Calculation/Nonlinear FK Force Variant Subsystem/With Nonlinear FroudeKrylov Force ==
  Time : Inport
  Displacement : Inport  Port=2
  WaveElv : Inport  Port=3
  Add : Sum  Inputs=+-
  Center of Gravity : Constant  Value=body.hydroData.properties.centerGravity
  Center of Gravity1 : Constant  Value=body.hydroData(1).properties.centerGravity
  Constant : Constant  Value=zeros(1,body.dof-body.gbmDOF-3)
  Constant1 : Constant  Value=zeros(body.gbmDOF,1)
  Deep Water Flag : Constant  Value=waves.deepWater
  Diffraction and Excitation Forces : MATLAB Function  TreatAsAtomicUnit=on
  Frequency Spacing : Constant  Value=waves.dOmega
  Gravity : Constant  Value=simu.gravity
  Mux : Mux  Inputs=2
  Mux1 : Mux  Inputs=2
  STL Areas : Constant  Value=body.geometry.area
  STL Centers : Constant  Value=body.geometry.center
  STL Normal Vectors : Constant  Value=body.geometry.norm
  Selector : Selector  InputPortWidth=body.dof  IndexOptions=Index vector (dialog)  Indices=[1:6]  OutputSizes=1
  To Workspace : ToWorkspace  VariableName=body1_wavenonlinearpressure_out  SaveFormat=Structure With Time  SampleTime=-1
      settings: Decimation=round(simu.dtOut/simu.dt,0)
  To Workspace1 : ToWorkspace  VariableName=body1_wavelinearpressure_out  SaveFormat=Structure With Time  SampleTime=-1
      settings: Decimation=round(simu.dtOut/simu.dt,0)
  Water Density : Constant  Value=simu.rho
  Water Depth : Constant  Value=waves.waterDepth
  Wave Amplitude : Constant  Value=waves.amplitude
  Wave Direction : Constant  Value=waves.direction
  Wave Frequency : Constant  Value=waves.omega
  Wave Number : Constant  Value=waves.wavenumber
  Wave Random Phase : Constant  Value=waves.phase
  Wave Spread : Constant  Value=waves.spread
  Wave Type Number : Constant  Value=waves.typeNum
  Nonlinear Excitation : Outport
  wires:
  Wave Direction/1 -> Diffraction and Excitation Forces/3(direction)
  STL Areas/1 -> Diffraction and Excitation Forces/7(area)
  Diffraction and Excitation Forces/2(wp) -> To Workspace/1
  Diffraction and Excitation Forces/3(wpMeanFS) -> To Workspace1/1
  Displacement/1 -> Selector/1
  Constant/1 -> Mux/2
  Center of Gravity/1 -> Mux/1  "cg"
  Mux/1 -> Add/2
  Add/1 -> Diffraction and Excitation Forces/1(x)  "x_cg"
  Deep Water Flag/1 -> Diffraction and Excitation Forces/15(deepWater)
  Wave Random Phase/1 -> Diffraction and Excitation Forces/19(phaseRand)
  Water Depth/1 -> Diffraction and Excitation Forces/14(wDepth)
  Wave Number/1 -> Diffraction and Excitation Forces/16(k)
  Wave Type Number/1 -> Diffraction and Excitation Forces/17(typeNum)
  Frequency Spacing/1 -> Diffraction and Excitation Forces/13(dw)
  Wave Frequency/1 -> Diffraction and Excitation Forces/12(w)
  Wave Amplitude/1 -> Diffraction and Excitation Forces/11(AH)
  Time/1 -> Diffraction and Excitation Forces/18(t)
  WaveElv/1 -> Diffraction and Excitation Forces/2(elv)
  STL Normal Vectors/1 -> Diffraction and Excitation Forces/6(tnorm)
  Water Density/1 -> Diffraction and Excitation Forces/8(rho)
  Gravity/1 -> Diffraction and Excitation Forces/9(g)
  Diffraction and Excitation Forces/1(f) -> Mux1/1
  Center of Gravity1/1 -> Diffraction and Excitation Forces/10(cg)
  Selector/1 -> Add/1
  Constant1/1 -> Mux1/2
  Mux1/1 -> Nonlinear Excitation/1
  STL Centers/1 -> Diffraction and Excitation Forces/5(center)
  Wave Spread/1 -> Diffraction and Excitation Forces/4(spread)

== system WECSim_Lib_Body_Elements/Flex Body/Wave Radiation Forces Calculation/Wave Radiation Forces Calculation/SS CI and Constant-Damping-CoeVariant Subsystem/Constant Coefficients ==
  note: F = damping * velocity
  velocity : Inport
  Bus Selector : BusSelector  OutputSignals=fDamping
  Product : Product  Multiplication=Matrix(*)
  Out1 : Outport
  wires:
  Bus Selector/1 -> Product/1  "<fDamping>"
  [body1_hydroForce] -> Bus Selector/1
  velocity/1 -> Product/2
  Product/1 -> Out1/1  "F_Single Frequency"

== system WECSim_Lib_Body_Elements/Flex Body/Wave Radiation Forces Calculation/Wave Radiation Forces Calculation/SS CI and Constant-Damping-CoeVariant Subsystem/Convolution Integral Calculation ==
  velocity : Inport
  Convolution Variant Subsystem : Subsystem  Variant=on  VariantControl=Subsystem
  Rate Transition : RateTransition
  Reshape : Reshape
  Out1 : Outport
  wires:
  Convolution Variant Subsystem/1(Frad) -> Rate Transition/1
  velocity/1 -> Convolution Variant Subsystem/1(velocity)
  Rate Transition/1 -> Reshape/1
  Reshape/1 -> Out1/1

== system WECSim_Lib_Body_Elements/Flex Body/Wave Radiation Forces Calculation/Wave Radiation Forces Calculation/SS CI and Constant-Damping-CoeVariant Subsystem/FIR Filter Calculation ==
  velocity : Inport
  FIR Filter Matrix : Subsystem  mask{B2B=simu.b2b, body=body}
      mask prompts: body "bodyClass"
      mask init:
      | if exist('body','var')
      |     TotalRows = body.dof;
      |     
      |     cb = gcb;
      |     
      |     set_param([cb '/Mux'],...
      |                'Inputs',sprintf('%d',TotalRows));
      |     
      |     set_param([cb '/FIR_filter_row'],...
      |                'position',[0, 100, 200, 140]);
      |     
      |     set_param([cb '/FIR_filter_row'],...
      |                'rowNo', '1');
      |     
      |     try
      |     add_line(cb,...
      |             ['velocity','/1'], ...    
      |             'FIR_filter_row/1',... 
      |             'autorouting','on');
      |     catch
      |     end
      |     
      |     try
      |     add_line(cb,...
      |             ['FIR_filter_row','/1'], ...    
      |             'Mux/1',... 
      |             'autorouting','on');
      |     catch
      |     end
      |     
      |     for i = 2:TotalRows
      |         add_block([cb,'/FIR_filter_row'],[cb,'/FIR_filter_row',num2str(i)], 'MakeNameUnique','off');
      |         set_param([cb '/FIR_filter_row',num2str(i)],...
      |                    'position',[0, 100*i, 200, 40 + 100*i]);
      |         set_param([cb '/FIR_filter_row',num2str(i)],...
      |                    'rowNo', num2str(i));
      |         add_line(cb,...
      |                 ['velocity','/1'], ...    
      |                 ['FIR_filter_row',num2str(i),'/1'],... 
      |                 'autorouting','on');
      |         add_line(cb,...
      |                 ['FIR_filter_row',num2str(i),'/1'], ...    
      |                 ['Mux/',num2str(i)],... 
      |                 'autorouting','on');
      |     end
      | end
  Rate Transition : RateTransition  OutPortSampleTime=simu.cicDt
  Rate Transition1 : RateTransition  OutPortSampleTime=simu.cicDt
  Out1 : Outport
  wires:
  Rate Transition1/1 -> Out1/1
  Rate Transition/1 -> FIR Filter Matrix/1(velocity)
  FIR Filter Matrix/1(Out1) -> Rate Transition1/1
  velocity/1 -> Rate Transition/1

== system WECSim_Lib_Body_Elements/Flex Body/Wave Radiation Forces Calculation/Wave Radiation Forces Calculation/SS CI and Constant-Damping-CoeVariant Subsystem/State-Space Calculation  ==
  note: Calculate the radiation damping based on the state space formulation. Coefficients are defined in body.hydroForce.ssRadf
  velocity : Inport
  State-Space : StateSpace  A=body.hydroForce.hf1.ssRadf.A  B=body.hydroForce.hf1.ssRadf.B  C=body.hydroForce.hf1.ssRadf.C  D=body.hydroForce.hf1.ssRadf.D  InitialCondition=0
  Out1 : Outport
  wires:
  State-Space/1 -> Out1/1
  velocity/1 -> State-Space/1  "x"

== system WECSim_Lib_Body_Elements/Rigid Body/Hydrodynamic Body/B2B Subsystem/B2B/CrossCoupling ==
  note: CrossCoupling block is updated by its mask initialization, which is only called on when a simulation is run. 'From' blocks are automatically created and connected based on the number of bodies in the simulation.
  Mux1 : Mux  Inputs=2
  Mux2 : Mux  Inputs=2
  Transport Delay1 : TransportDelay  DelayTime=10e-8
  Transport Delay2 : TransportDelay  DelayTime=1e-07
  vel : Outport
  acc : Outport  Port=2
  wires:
  [vel1] -> Mux1/1
  Mux1/1 -> vel/1
  [acc1] -> Transport Delay1/1
  Mux2/1 -> acc/1
  Transport Delay1/1 -> Mux2/1
  [vel2] -> Mux1/2
  [acc2] -> Transport Delay2/1
  Transport Delay2/1 -> Mux2/2
